simulink model "mu_linear_sim"  (R2026a)
settings: Solver=VariableStepAuto
InitFcn:
  | seaDir=fileparts(get_param(bdroot,'FileName'));if isfile(fullfile(seaDir,'..','collaudo_simulink.m')),addpath(fullfile(seaDir,'..'));else,addpath(fullfile(seaDir,'..','..','File_di_Funzioni_Progetto-Accorpati'));end;collaudo_simulink(bdroot);
undefined symbols (not defined in the file): Aplant, Bplant, Cplant, Dplant, x0plant
libraries: cstblocks_lti x1
settings Model: Creator=rebec  LastModifiedBy=rebec

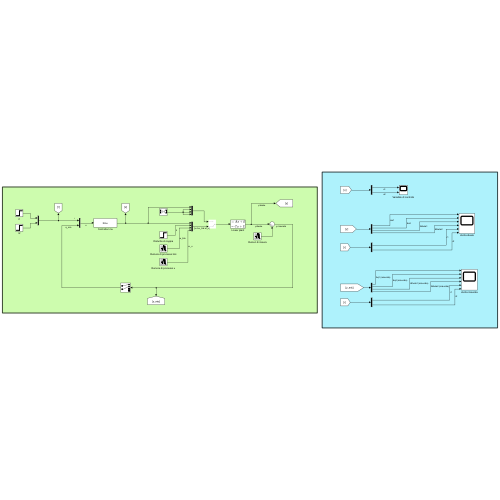
[thumbnail: Simulink's stored preview of the top-level diagram]
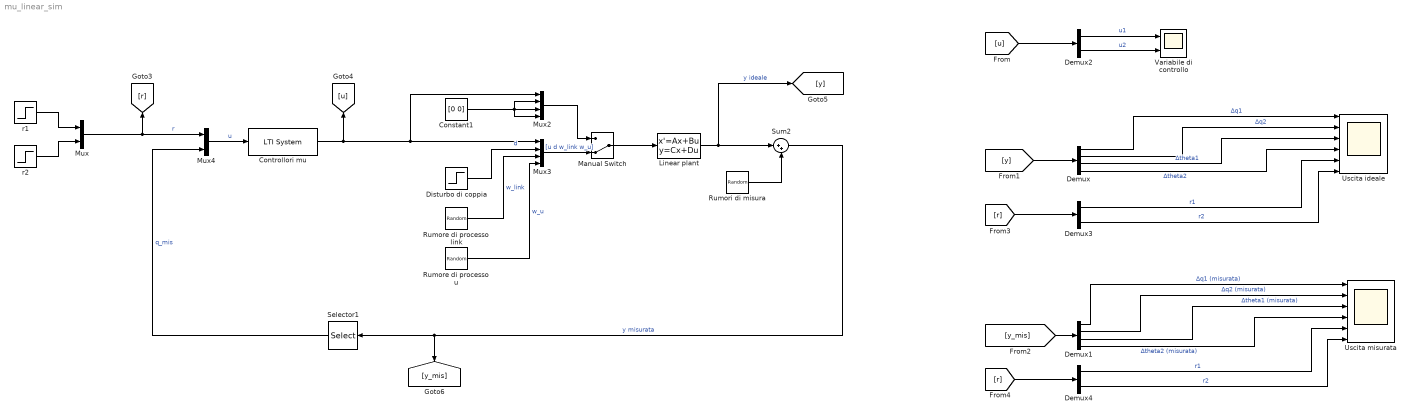
== system mu_linear_sim ==
  Constant1 : Constant  Value=[0 0]
  Controllori mu : cstblocks_lti/LTI System  sys=Kmu  IC=[]  PadeOrder=0
      settings: LibrarySourceBlock=cstblocks/LTI System
  Demux : Demux
  Demux1 : Demux
  Demux2 : Demux  Outputs=2
  Demux3 : Demux  Outputs=2
  Demux4 : Demux  Outputs=2
  Disturbo di coppia : Step  Time=[1 1]  InitialValue=[0 0]  FinalValue=[0.5 0]  SampleTime=0
  Linear plant : StateSpace  A=Aplant  B=Bplant  C=Cplant  D=Dplant  InitialCondition=x0plant
  Manual Switch : ManualSwitch  CurrentSetting=0
  Mux : Mux  Inputs=2
  Mux2 : Mux
  Mux3 : Mux
  Mux4 : Mux  Inputs=2
  Rumore di processo link : RandomNumber  Mean=[0 0]  Variance=[0.01 0.01]  Seed=20260826  SampleTime=0.002
  Rumore di processo u : RandomNumber  Mean=[0 0]  Variance=[0.01 0.01]  Seed=20260826  SampleTime=0.002
  Rumori di misura : RandomNumber  Mean=[0 0 0 0]  Variance=[(0.05*pi/180)^2 (0.05*pi/180)^2 (0.05*pi/180)^2 (0.05*pi/180)^2]  Seed=20260826  SampleTime=0.002
  Selector1 : Selector  InputPortWidth=4  IndexOptions=Index vector (dialog)  Indices=[1 2]  OutputSizes=1
  Sum2 : Sum  Inputs=|++
  Uscita ideale : Scope  NumInputPorts=6
      settings: Title=y (uscita ideale)  ActiveDisplayYMinimum=-0.088271118920575181  ActiveDisplayYMaximum=0.23303114019935003
  Uscita misurata : Scope  NumInputPorts=6
      settings: Title=y (uscita ideale)  ActiveDisplayYMinimum=-0.11442029066688837  ActiveDisplayYMaximum=0.16914890182413583
  Variabile di controllo : Scope  NumInputPorts=2
      settings: ActiveDisplayYMinimum=-0.70674754070580625  ActiveDisplayYMaximum=0.0520180612501398  DataLoggingVariableName=ScopeData2
  r1 : Step  FinalValue=5*pi/180  SampleTime=0
  r2 : Step  FinalValue=0  SampleTime=0
  wires:
  Mux/1 -> Mux4/1, [r]  "r"
  Constant1/1 -> Mux2/2, Mux2/4, Mux2/3
  Rumore di processo link/1 -> Mux3/3  "w_link"
  r2/1 -> Mux/2
  Disturbo di coppia/1 -> Mux3/2  "d"
  Manual Switch/1 -> Linear plant/1
  Mux4/1 -> Controllori mu/1  "u"
  Rumore di processo u/1 -> Mux3/4  "w_u"
  Sum2/1 -> [y_mis], Selector1/1  "y misurata"
  r1/1 -> Mux/1
  Mux2/1 -> Manual Switch/1
  Linear plant/1 -> [y], Sum2/1  "y ideale"
  Mux3/1 -> Manual Switch/2  "[u d w_link w_u]"
  Selector1/1 -> Mux4/2  "q_mis"
  Controllori mu/1 -> Mux2/1, Mux3/1, [u]
  [y_mis] -> Demux1/1
  Demux4/2 -> Uscita misurata/6  "r2"
  Demux1/4 -> Uscita misurata/4  "Δtheta2 (misurata)"
  [r] -> Demux3/1
  Demux1/2 -> Uscita misurata/2  "Δq2 (misurata)"
  Demux4/1 -> Uscita misurata/5  "r1"
  [r] -> Demux4/1
  Demux/3 -> Uscita ideale/3  "Δtheta1"
  Demux/4 -> Uscita ideale/4  "Δtheta2"
  [y] -> Demux/1
  Demux/1 -> Uscita ideale/1  "Δq1"
  Demux/2 -> Uscita ideale/2  "Δq2"
  Demux2/1 -> Variabile di controllo/1  "u1"
  Demux3/2 -> Uscita ideale/6  "r2"
  Demux1/3 -> Uscita misurata/3  "Δtheta1 (misurata)"
  Demux3/1 -> Uscita ideale/5  "r1"
  Demux2/2 -> Variabile di controllo/2  "u2"
  [u] -> Demux2/1
  Demux1/1 -> Uscita misurata/1  "Δq1 (misurata)"
  Rumori di misura/1 -> Sum2/2
